simulink library "MK_H"  (R2026a)
settings: Solver=VariableStepAuto
undefined symbols (not defined in the file): K, tau, xi, y_0, z_0
settings Model: Creator=Szalay  LastModifiedBy=Szalay

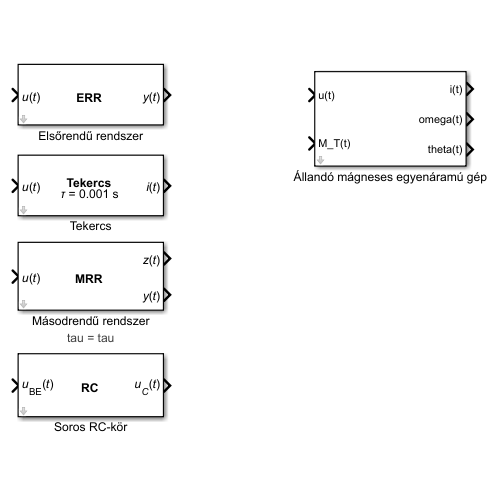
[thumbnail: Simulink's stored preview of the top-level diagram]
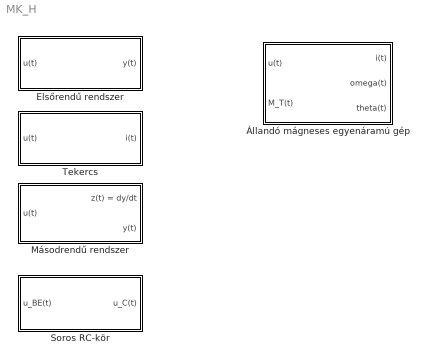
== system MK_H ==
  Elsőrendű rendszer : Subsystem  mask(Elsőrendű rendszer){K=1, tau=tau, y_0=2.5}
      mask prompts: K "Állandósult állapoti erősítés"; tau "Időállandó"; y_0 "A kimenet kezdeti értéke"
      mask help: A lineáris elsőrendű rendszer modellje.
      mask DialogControl ParameterGroupVar Prompt: Rendszerparaméterek
      mask DialogControl Container3 Prompt: Kezdeti érték
      mask Display:
      | % Csatlakozók
      | port_label('input', 1, '{\itu}({\itt})', 'texmode', 'on')
      | port_label('output', 1, '{\ity}({\itt})', 'texmode', 'on');
      | 
      | % Felirat
      | text(0.5, 0.5, '{\bfERR}', ...
      |     'HorizontalAlignment', 'center', ...
      |     'texmode', 'on' ...
      |     );
  Másodrendű rendszer : Subsystem  mask(Másodrendű rendszer){K=K, tau=tau, xi=xi, y_0=y_0, z_0=z_0}
      mask prompts: K "Állandósult állapoti erősítés"; tau "Időállandó (s)"; xi "Csillapítási tényező"; y_0 "Kezdeti y"; z_0 "Kezdeti z"
      mask help: A közönséges lineáris másodfokú differenciálegyenlet megvalósítása.
      settings: AttributesFormatString=tau = %<tau>
      mask DialogControl ParameterGroupVar Prompt: Rendszerparaméterek
      mask DialogControl Container3 Prompt: Kezdeti értékek
      mask Display:
      | % Csatlakozók
      | port_label('input', 1, '{\itu}({\itt})', 'texmode', 'on');
      | port_label('output', 1, '{\itz}({\itt})', 'texmode', 'on');
      | port_label('output', 2, '{\ity}({\itt})', 'texmode', 'on');
      | 
      | % Felirat
      | text(0.5, 0.5, '{\bfMRR}', ...
      |     'HorizontalAlignment', 'center', ...
      |     'Interpreter', 'tex' ...
      |     );
  Soros RC-kör : Subsystem  mask(Soros RC-kör){R=1, C=1e-6, u_C0=0}
      mask prompts: R "Ellenállás"; C "Kapacitás"; u_C0 "A kapacitás kezdeti feszültsége"
      mask help: Egyszerű soros RC-kör.
      mask DialogControl ParameterGroupVar Prompt: Modellparaméterek
      mask DialogControl Container3 Prompt: Kezdeti érték
      mask Display:
      | % Csatlakozók
      | port_label('input', 1, '{\itu}_{BE}({\itt})', 'texmode', 'on');
      | port_label('output', 1, '{\itu}_{\itC}({\itt})', 'texmode', 'on');
      | 
      | % Felirat
      | text(0.5, 0.5, '{\bfRC}', ...
      |     'HorizontalAlignment', 'center', 'Interpreter', 'tex' ...
      |     );
  Tekercs : Subsystem  mask(Tekercs){R=1, L=1e-3, i_0=0}
      mask prompts: R "Ellenállás"; L "Öninduktivitás"; i_0 "Kezdeti áramerősség"
      mask help: Soros RL-tag alapú lineáris tekercsmodell.
      mask DialogControl ParameterGroupVar Prompt: Modellparaméterek
      mask DialogControl Container3 Prompt: Kezdeti érték
      mask Display:
      | % Csatlakozók
      | port_label('input', 1, '{\itu}({\itt})', 'texmode', 'on')
      | port_label('output', 1, '{\iti}({\itt})', 'texmode', 'on');
      | 
      | % Időállandó
      | R = str2double(get_param(gcb, 'R'));
      | L = str2double(get_param(gcb, 'L'));
      | 
      | tau = L/R;
      | 
      | % Felirat
      | text(0.5, 0.5, [ ...
      |     '{\bfTekercs}', newline, '{\it\tau} = ', sprintf('%g', tau) ' s' ...
      |     ], ...
      |     'HorizontalAlignment', 'center', ...
      |     'texmode', 'on' ...
      |     );
  Állandó mágneses egyenáramú gép : Subsystem  mask(ÁMEG){R=0.079, L=26e-6, k_T=13.7e-3, k_E=13.7e-3, J=99.5e-7, B=5.1493e-6, i_0=0, omega_0=0, theta_0=0}
      mask prompts: R "Ellenállás (Ohm)"; L "Induktivitás (H)"; k_T "Nyomatékállandó (Nm/A)"; k_E "Feszültségállandó (Vs/rad)"; J "Tehetetlenségi nyomaték (kgm^2)"; B "Forgási súrlódási együttható (Nms/rad)"; i_0 "Kezdeti áramerősség (A)"; omega_0 "Kezdeti szögsebesség (rad/s)"; theta_0 "Kezdeti szöghelyzet (rad)"
      mask help: Az állandó mágneses egyenáramú gép modellje a Maxon DCX 35L 12 V-os változata alapján felparaméterezve.
      mask DialogControl ParameterGroupVar Prompt: Villamos áramköri részrendszer
      mask DialogControl Container3 Prompt: Gépállandók
      mask DialogControl Container4 Prompt: Forgó részrendszer
      mask DialogControl Container5 Prompt: Kezdeti értékek

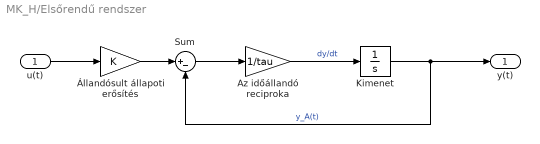
== system MK_H/Elsőrendű rendszer ==
  u(t) : Inport
  Az időállandó reciproka : Gain  Gain=1/tau
  Kimenet : Integrator  InitialCondition=y_0
  Sum : Sum  Inputs=|+-
  Állandósult állapoti erősítés : Gain  Gain=K
  y(t) : Outport
  wires:
  u(t)/1 -> Állandósult állapoti erősítés/1
  Kimenet/1 -> y(t)/1, Sum/2  "y_A(t)"
  Az időállandó reciproka/1 -> Kimenet/1  "dy/dt"
  Sum/1 -> Az időállandó reciproka/1
  Állandósult állapoti erősítés/1 -> Sum/1

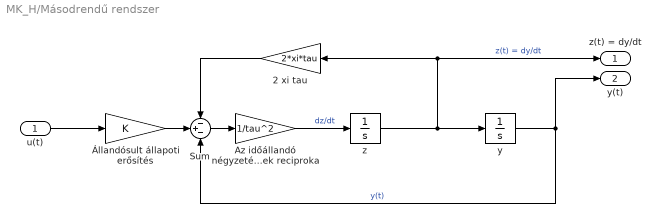
== system MK_H/Másodrendű rendszer ==
  u(t) : Inport
  2 xi tau : Gain  Gain=2*xi*tau
  Az időállandó négyzetének reciproka : Gain  Gain=1/tau^2
  Sum : Sum  Inputs=-+-
  y : Integrator  InitialCondition=y_0
  z : Integrator  InitialCondition=z_0
  Állandósult állapoti erősítés : Gain  Gain=K
  z(t) = dy/dt : Outport
  y(t) : Outport  Port=2
  wires:
  Állandósult állapoti erősítés/1 -> Sum/2
  2 xi tau/1 -> Sum/1
  u(t)/1 -> Állandósult állapoti erősítés/1
  Sum/1 -> Az időállandó négyzetének reciproka/1
  Az időállandó négyzetének reciproka/1 -> z/1  "dz/dt"
  y/1 -> Sum/3, y(t)/1  "y(t)"
  z/1 -> y/1, 2 xi tau/1, z(t) = dy/dt/1  "z(t) = dy/dt"

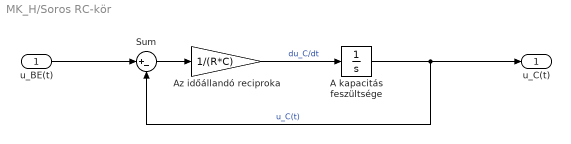
== system MK_H/Soros RC-kör ==
  u_BE(t) : Inport
  A kapacitás feszültsége : Integrator  InitialCondition=u_C0
  Az időállandó reciproka : Gain  Gain=1/(R*C)
  Sum : Sum  Inputs=|+-
  u_C(t) : Outport
  wires:
  u_BE(t)/1 -> Sum/1
  Az időállandó reciproka/1 -> A kapacitás feszültsége/1  "du_C/dt"
  A kapacitás feszültsége/1 -> u_C(t)/1, Sum/2  "u_C(t)"
  Sum/1 -> Az időállandó reciproka/1

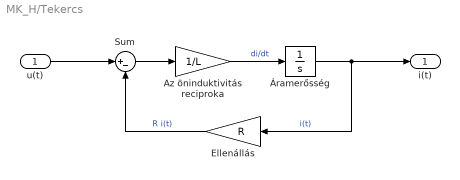
== system MK_H/Tekercs ==
  u(t) : Inport
  Az öninduktivitás reciproka : Gain  Gain=1/L
  Ellenállás : Gain  Gain=R
  Sum : Sum  Inputs=|+-
  Áramerősség : Integrator  InitialCondition=i_0
  i(t) : Outport
  wires:
  Az öninduktivitás reciproka/1 -> Áramerősség/1  "di/dt"
  Ellenállás/1 -> Sum/2  "R i(t)"
  Áramerősség/1 -> Ellenállás/1, i(t)/1  "i(t)"
  Sum/1 -> Az öninduktivitás reciproka/1
  u(t)/1 -> Sum/1

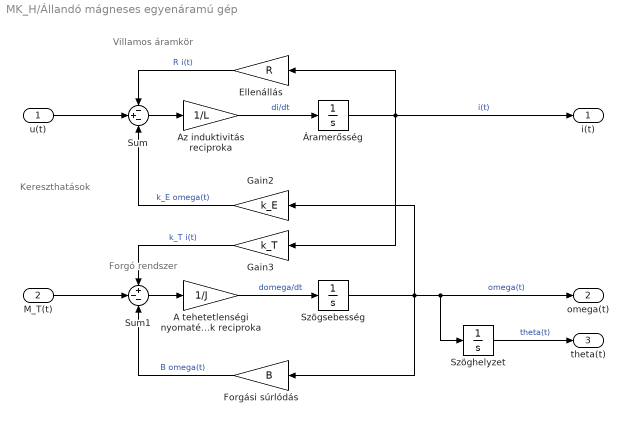
== system MK_H/Állandó mágneses egyenáramú gép ==
  note: Kereszthatások
  note: Forgó rendszer
  note: Villamos áramkör
  u(t) : Inport
  M_T(t) : Inport  Port=2
  A tehetetlenségi nyomaték reciproka : Gain  Gain=1/J
  Az induktivitás reciproka : Gain  Gain=1/L
  Ellenállás : Gain  Gain=R
  Forgási súrlódás : Gain  Gain=B
  Gain2 : Gain  Gain=k_E
  Gain3 : Gain  Gain=k_T
  Sum : Sum  Inputs=-+-
  Sum1 : Sum  Inputs=+--
  Szöghelyzet : Integrator  InitialCondition=theta_0
  Szögsebesség : Integrator  InitialCondition=omega_0
  Áramerősség : Integrator  InitialCondition=i_0
  i(t) : Outport
  omega(t) : Outport  Port=2
  theta(t) : Outport  Port=3
  wires:
  Sum/1 -> Az induktivitás reciproka/1
  Áramerősség/1 -> i(t)/1, Gain3/1, Ellenállás/1  "i(t)"
  Ellenállás/1 -> Sum/1  "R i(t)"
  Sum1/1 -> A tehetetlenségi nyomaték reciproka/1
  Szögsebesség/1 -> omega(t)/1, Szöghelyzet/1, Gain2/1, Forgási súrlódás/1  "omega(t)"
  Gain2/1 -> Sum/3  "k_E omega(t)"
  Az induktivitás reciproka/1 -> Áramerősség/1  "di/dt"
  A tehetetlenségi nyomaték reciproka/1 -> Szögsebesség/1  "domega/dt"
  Forgási súrlódás/1 -> Sum1/3  "B omega(t)"
  Gain3/1 -> Sum1/1  "k_T i(t)"
  u(t)/1 -> Sum/2
  M_T(t)/1 -> Sum1/2
  Szöghelyzet/1 -> theta(t)/1  "theta(t)"
